simulink model "servo_transfer_cell"  (R2026a)
settings: Solver=ode4  StopTime=16  FixedStep=0.002
model workspace (MAT data in the model file):
  brakeDamping = 240
  commandData = [0 0.01 0.02 0.03 0.04 0.05 0.06 0.07 0.08 0.09 0.1 0.11 ... (17611 elements, 1601x11)]
  params = [0.01 8 6 1.5 35 0.45 0.8 2 75 110 10 0.65 ... (18 elements, 1x18)]
  plantCoulomb = 1.5
  plantMass = 8
  plantViscous = 6
(part 2 of 2)

== matlab function servo_transfer_cell/Servo ==
  data: x input; force output; v input; target input; state input; cmd input; p input; vref output; brake output
function [force,vref,brake] = servo(x,v,target,state,cmd,p)
persistent mem
if isempty(mem), mem=zeros(1,2); end
[force,vref,brake,mem]=cellctl.servo_step(x,v,target,state,cmd(10),p,mem);
end

== matlab function servo_transfer_cell/Sequence ==
  data: x input; state output; v input; cmd input; p input; target output; alarm output; cycles output
function [state,target,alarm,cycles] = sequence(x,v,cmd,p)
persistent mem
if isempty(mem), mem=zeros(1,8); end
[state,target,alarm,cycles,mem]=cellctl.sequence_step(x,v,cmd,p,mem);
end

== matlab function servo_transfer_cell/LoadAndFriction ==
  data: v input; loss output; cmd input; brake input; p input
function loss=losses(v,cmd,brake,p)
loss=p(3)*v+p(4)*tanh(v/0.01)+cmd(8)+brake*p(18)*v;
end
